simulink model "SRF_2DOF_Method"  (R2024b)
settings: Solver=VariableStepAuto  StartTime=0.0  StopTime=0.6  RelTol=1e-3
undefined symbols (not defined in the file): alpha, beta, ti
libraries: spsSeriesRLCBranchLib x6, spsMosfetLib x6, spsThreePhaseVIMeasurementLib x3, spsThreePhaseSeriesRLCBranchLib x2, eeGeneralControl x2, slpidlib x2, spsabctodq0Lib x2, spsCurrentMeasurementLib x1, spsGroundLib x1, spsdq0toabcLib x1, spsThreePhaseBreakerLib x1, spsThreePhaseSourceLib x1
settings Model: Creator=ASUS  LastModifiedBy=ASUS
settings DataIOCC: SaveFormat=StructureWithTime  ReturnWorkspaceOutputs=off

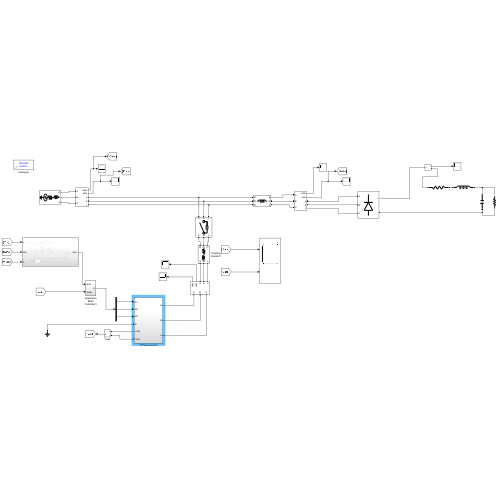
[thumbnail: Simulink's stored preview of the top-level diagram]
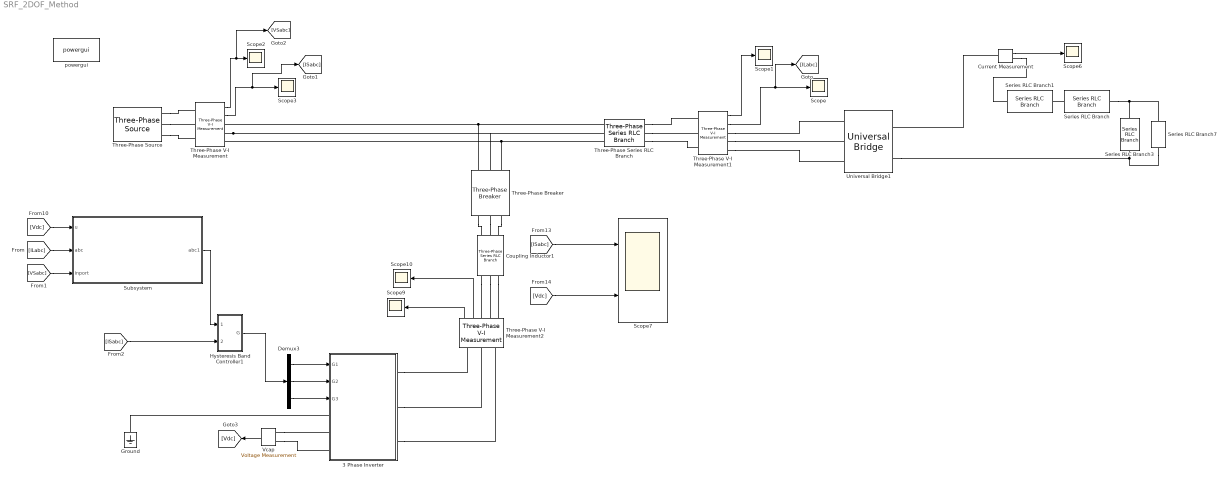
== system SRF_2DOF_Method ==
  3 Phase Inverter : Subsystem
  Coupling Inductor1 : spsThreePhaseSeriesRLCBranchLib/Three-Phase Series RLC Branch  LConnTagsString=A|B|C  RConnTagsString=A|B|C  BranchType=RL  Resistance=0.01  Inductance=3.5e-3  Capacitance=1e-6  Measurements=None
  Current Measurement : spsCurrentMeasurementLib/Current Measurement  PhasorSimulation=off  OutputType=Complex  PSBequivalent=0
  Demux3 : Demux  Outputs=3
  Ground : spsGroundLib/Ground  LConnTagsString=a
  Hysteresis Band Controller1 : Subsystem
  Scope{,1..3,6,9..10} (7 alike) : Scope
  Scope7 : Scope  NumInputPorts=2
  Series RLC Branch : spsSeriesRLCBranchLib/Series RLC Branch  LConnTagsString=__new0  RConnTagsString=__new0  BranchType=L  Resistance=50  Inductance=2e-6  SetiL0=off  InitialCurrent=0  Capacitance=1e-6  Setx0=off  InitialVoltage=0  Measurements=None
  Series RLC Branch1 : spsSeriesRLCBranchLib/Series RLC Branch  LConnTagsString=__new0  RConnTagsString=__new0  BranchType=R  Resistance=0.06  Inductance=1e-3  SetiL0=off  InitialCurrent=0  Capacitance=1e-6  Setx0=off  InitialVoltage=0  Measurements=None
  Series RLC Branch3 : spsSeriesRLCBranchLib/Series RLC Branch  LConnTagsString=__new0  RConnTagsString=__new0  BranchType=C  Resistance=50  Inductance=1e-3  SetiL0=off  InitialCurrent=0  Capacitance=3.63e-9  Setx0=off  InitialVoltage=0  Measurements=None
  Series RLC Branch7 : spsSeriesRLCBranchLib/Series RLC Branch  LConnTagsString=__new0  RConnTagsString=__new0  BranchType=R  Resistance=51.054  Inductance=1e-3  SetiL0=off  InitialCurrent=0  Capacitance=1e-6  Setx0=off  InitialVoltage=0  Measurements=None
  Subsystem : Subsystem
  Three-Phase Series RLC Branch : spsThreePhaseSeriesRLCBranchLib/Three-Phase Series RLC Branch  LConnTagsString=A|B|C  RConnTagsString=A|B|C  BranchType=L  Resistance=1  Inductance=1e-3  Capacitance=1e-6  Measurements=None
  Three-Phase V-I Measurement : spsThreePhaseVIMeasurementLib/Three-Phase V-I Measurement  VoltageMeasurement=phase-to-ground  SetLabelV=off  LabelV=Vabc  Vpu=off  VpuLL=off  CurrentMeasurement=yes  SetLabelI=off  LabelI=Iabc  Ipu=off  Pbase=100e6  Vbase=500e3  OutputType=Complex  PhasorSimulation=off  PSBequivalent=0
  Three-Phase V-I Measurement1 : spsThreePhaseVIMeasurementLib/Three-Phase V-I Measurement  VoltageMeasurement=phase-to-ground  SetLabelV=off  LabelV=Vabc  Vpu=off  VpuLL=off  CurrentMeasurement=yes  SetLabelI=off  LabelI=Iabc  Ipu=off  Pbase=100e6  Vbase=500e3  OutputType=Complex  PhasorSimulation=off  PSBequivalent=0
  Three-Phase V-I Measurement2 : spsThreePhaseVIMeasurementLib/Three-Phase V-I Measurement  VoltageMeasurement=phase-to-ground  SetLabelV=off  LabelV=Vabc  Vpu=off  VpuLL=off  CurrentMeasurement=yes  SetLabelI=off  LabelI=Iabc  Ipu=off  Pbase=100e6  Vbase=500e3  OutputType=Complex  PhasorSimulation=off  PSBequivalent=0
  Three-Phase Breaker : spsThreePhaseBreakerLib/Three-Phase Breaker  InitialState=open  SwitchA=on  SwitchB=on  SwitchC=on  SwitchTimes=[0.2 0.5]  External=off  BreakerResistance=0.01  SnubberResistance=1e6  SnubberCapacitance=inf  Measurements=None
  Three-Phase Source : spsThreePhaseSourceLib/Three-Phase Source  InternalConnection=Yg  VoltagePhases=off  Voltage=415  PhaseAngle=0  Voltage_phases=[25e3 25e3 25e3]/sqrt(3)  PhaseAngles_phases=[0 -120 +120]  Frequency=50  NonIdealSource=on  SpecifyImpedance=off  Resistance=0.86  Inductance=1e-4  ShortCircuitLevel=100e6  BaseVoltage=25e3  XRratio=7  BusType=swing  Pref=10e3  Qref=0  Prefabc=[10e3, 10e3, 10e3]  Qrefabc=[0, 0, 0]  Qmin=-inf  Qmax=inf
  Universal Bridge1 : spsUniversalBridgeLib/Universal Bridge  Arms=3  SnubberResistance=1e5  SnubberCapacitance=inf  Device=Diodes  Ron=1e-3  Lon=0  ForwardVoltages="[  0  0  ]"  ForwardVoltage=0  GTOparameters=[ 10e-6 , 20e-6 ]  IGBTparameters=[ 1e-6 , 2e-6 ]  Measurements=None  Measurements_2=None  converterType=Rectifier
  Vcap : spsVoltageMeasurementLib/Voltage Measurement  PhasorSimulation=off  OutputType=Complex  PSBequivalent=0
  powergui : spspowerguiLib/powergui  Priority=1  SimulationMode=Discrete  SampleTime=30e-07  frequency=60  Iterations=50  frequencyindice=0  Pbase=100e6  ErrMax=1e-4  UnitsV=kV  UnitsW=MW  buscounter=0  FunctionMessages=off  echomessages=off  EnableUseOfTLC=off  CurrentSourceSwitches=off  DisableSnubberDevices=off  DisableRonSwitches=off  DisableVfSwitches=off  DisplayEquations=off  AutomaticDiscreteSolvers=off  SolverType=Tustin/Backward Euler (TBE)  Interpol=off  ExternalGateDelay=off  methode=off  Ts=100  x0status=blocks  SPID=on  SwTol=0  HookPort=off  NonlinearTolerance=1e-4  nMaxIteration=100  ContinueOnMaxIteration=off  RestoreLinks=warning  ResistiveCurrentMeasurement=off  Frange=[0:2:500]  Ylog=off  Xlog=on  ShowGrid=off  save=off  variable=ZData  structure=0  ZoomFFT=off  StartTime=0.0  cycles=1  DisplayStyle=1  fundamental=60  FreqAxis=off  MaxFrequency=1000  frequencyindicesteady=1  RmsSteady=1  display=off
  wires:
  Demux3/3 -> 3 Phase Inverter/3(G3)
  Current Measurement/1 -> Scope6/1
  [Vdc] -> Scope7/2
  Three-Phase V-I Measurement/2 -> [ISabc], Scope3/1
  Three-Phase V-I Measurement1/2 -> [ILabc], Scope/1
  Demux3/2 -> 3 Phase Inverter/2(G2)
  Three-Phase V-I Measurement1/1 -> Scope1/1
  Three-Phase V-I Measurement/1 -> [VSabc], Scope2/1
  Hysteresis Band Controller1/1(G) -> Demux3/1
  [ISabc] -> Hysteresis Band Controller1/2(ISabc)
  Three-Phase V-I Measurement2/2 -> Scope10/1
  [ISabc] -> Scope7/1
  Demux3/1 -> 3 Phase Inverter/1(G1)
  Vcap/1 -> [Vdc]
  Three-Phase V-I Measurement2/1 -> Scope9/1
  [VSabc] -> Subsystem/3(Inport)
  [Vdc] -> Subsystem/1(u)
  [ILabc] -> Subsystem/2(abc)
  Subsystem/1(abc1) -> Hysteresis Band Controller1/1(Isref)
  connections:
  Universal Bridge1/RConn2 -- Series RLC Branch3/RConn1 -- Series RLC Branch7/RConn1
  Three-Phase Breaker/RConn1 -- Three-Phase V-I Measurement/RConn1 -- Three-Phase Series RLC Branch/LConn1
  Series RLC Branch/RConn1 -- Series RLC Branch3/LConn1 -- Series RLC Branch7/LConn1
  Three-Phase Breaker/RConn3 -- Three-Phase V-I Measurement/RConn3 -- Three-Phase Series RLC Branch/LConn3
  Three-Phase V-I Measurement/RConn2 -- Three-Phase Series RLC Branch/LConn2 -- Three-Phase Breaker/RConn2
  Three-Phase Series RLC Branch/RConn2 -- Three-Phase V-I Measurement1/LConn2
  Three-Phase Source/RConn2 -- Three-Phase V-I Measurement/LConn2
  Three-Phase Series RLC Branch/RConn1 -- Three-Phase V-I Measurement1/LConn1
  3 Phase Inverter/RConn3 -- Three-Phase V-I Measurement2/LConn3
  Coupling Inductor1/RConn2 -- Three-Phase V-I Measurement2/RConn2
  3 Phase Inverter/LConn1 -- Ground/LConn1
  Three-Phase Series RLC Branch/RConn3 -- Three-Phase V-I Measurement1/LConn3
  Vcap/LConn1 -- 3 Phase Inverter/LConn2
  Coupling Inductor1/RConn3 -- Three-Phase V-I Measurement2/RConn3
  3 Phase Inverter/RConn2 -- Three-Phase V-I Measurement2/LConn2
  Three-Phase Breaker/LConn2 -- Coupling Inductor1/LConn2
  Three-Phase Source/RConn1 -- Three-Phase V-I Measurement/LConn1
  Current Measurement/LConn1 -- Universal Bridge1/RConn1
  Three-Phase V-I Measurement1/RConn1 -- Universal Bridge1/LConn1
  Three-Phase V-I Measurement1/RConn2 -- Universal Bridge1/LConn2
  Three-Phase V-I Measurement1/RConn3 -- Universal Bridge1/LConn3
  Three-Phase Source/RConn3 -- Three-Phase V-I Measurement/LConn3
  Three-Phase Breaker/LConn3 -- Coupling Inductor1/LConn3
  Coupling Inductor1/RConn1 -- Three-Phase V-I Measurement2/RConn1
  Vcap/LConn2 -- 3 Phase Inverter/LConn3
  Current Measurement/RConn1 -- Series RLC Branch1/RConn1
  3 Phase Inverter/RConn1 -- Three-Phase V-I Measurement2/LConn1
  Three-Phase Breaker/LConn1 -- Coupling Inductor1/LConn1
  Series RLC Branch/LConn1 -- Series RLC Branch1/LConn1

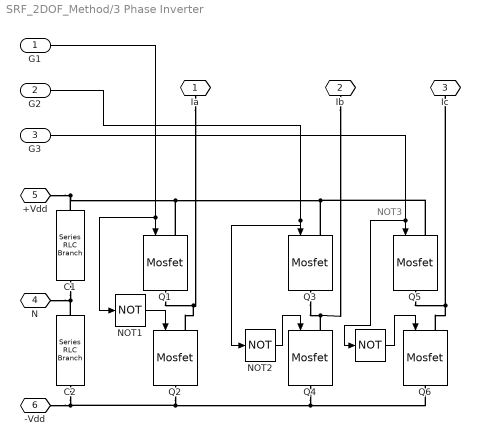
== system SRF_2DOF_Method/3 Phase Inverter ==
  note: NOT3
  G1 : Inport
  G2 : Inport  Port=2
  G3 : Inport  Port=3
  " " : Logic  Operator=NOT  AllPortsSameDT=off  OutDataTypeStr=boolean
  C1 : spsSeriesRLCBranchLib/Series RLC Branch  LConnTagsString=__new0  RConnTagsString=__new0  BranchType=C  Resistance=1  Inductance=1e-3  SetiL0=off  InitialCurrent=0  Capacitance=4700e-6  Setx0=off  InitialVoltage=350  Measurements=None
  C2 : spsSeriesRLCBranchLib/Series RLC Branch  LConnTagsString=__new0  RConnTagsString=__new0  BranchType=C  Resistance=1  Inductance=1e-3  SetiL0=off  InitialCurrent=0  Capacitance=4700e-6  Setx0=off  InitialVoltage=350  Measurements=None
  NOT1 : Logic  Operator=NOT  AllPortsSameDT=off  OutDataTypeStr=boolean
  NOT2 : Logic  Operator=NOT  AllPortsSameDT=off  OutDataTypeStr=boolean
  Q{1..6} (6 alike) : spsMosfetLib/Mosfet  Ron=0.01  Lon=0  Rd=0.01  Vfd=0  IC=0  Rs=1e10  Cs=inf  Measurements=off
  Ia : PMIOPort  Side=Right
  Ib : PMIOPort  Port=2  Side=Right
  Ic : PMIOPort  Port=3  Side=Right
  N : PMIOPort  Port=4  Side=Left
  +Vdd : PMIOPort  Port=5  Side=Left
  -Vdd : PMIOPort  Port=6  Side=Left
  wires:
  NOT1/1 -> Q2/1
  NOT2/1 -> Q4/1
  " "/1 -> Q6/1
  G1/1 -> NOT1/1, Q1/1
  G2/1 -> Q3/1, NOT2/1
  G3/1 -> Q5/1, " "/1
  connections:
  Q1/RConn1 -- Ia/RConn1 -- Q2/LConn1
  Q3/RConn1 -- Ib/RConn1 -- Q4/LConn1
  Q2/RConn1 -- C2/RConn1 -- -Vdd/RConn1 -- Q4/RConn1 -- Q6/RConn1
  Q6/LConn1 -- Ic/RConn1 -- Q5/RConn1
  C1/LConn1 -- Q1/LConn1 -- Q5/LConn1 -- Q3/LConn1 -- +Vdd/RConn1
  N/RConn1 -- C1/RConn1 -- C2/LConn1

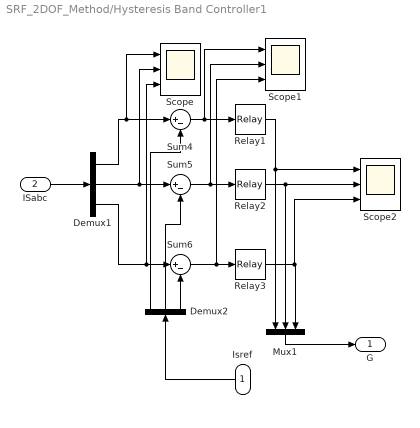
== system SRF_2DOF_Method/Hysteresis Band Controller1 ==
  Isref : Inport
  ISabc : Inport  Port=2
  Demux1 : Demux  Outputs=3
  Demux2 : Demux  Outputs=3
  Mux1 : Mux  Inputs=3
  Relay1 : Relay  OnSwitchValue=0.0001  OffSwitchValue=-0.0001  ZeroCross=off
  Relay2 : Relay  OnSwitchValue=0.0001  OffSwitchValue=-0.0001  ZeroCross=off
  Relay3 : Relay  OnSwitchValue=0.0001  OffSwitchValue=-0.0001  ZeroCross=off
  Scope : Scope  NumInputPorts=3
  Scope1 : Scope  NumInputPorts=3
  Scope2 : Scope  NumInputPorts=3
  Sum4 : Sum  Inputs=|+-
  Sum5 : Sum  Inputs=|+-
  Sum6 : Sum  Inputs=|+-
  G : Outport
  wires:
  Isref/1 -> Demux2/1
  ISabc/1 -> Demux1/1
  Mux1/1 -> G/1
  Sum4/1 -> Relay1/1, Scope1/1
  Demux2/1 -> Sum4/2
  Sum5/1 -> Relay2/1, Scope1/2
  Demux2/3 -> Sum6/2
  Demux1/3 -> Sum6/1, Scope/3
  Demux1/1 -> Sum4/1, Scope/1
  Sum6/1 -> Relay3/1, Scope1/3
  Demux1/2 -> Sum5/1, Scope/2
  Demux2/2 -> Sum5/2
  Relay2/1 -> Scope2/2, Mux1/2
  Relay1/1 -> Mux1/1, Scope2/1
  Relay3/1 -> Mux1/3, Scope2/3

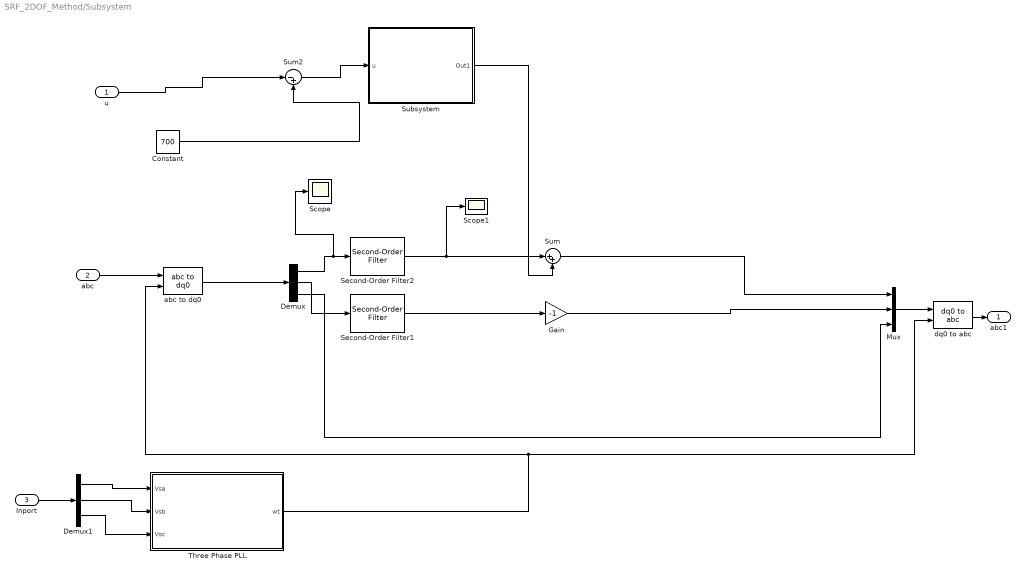
== system SRF_2DOF_Method/Subsystem ==
  u : Inport
  abc : Inport  Port=2
  Inport : Inport  Port=3
  Constant : Constant  Value=700
  Demux : Demux  Outputs=3
  Demux1 : Demux  Outputs=3
  Gain : Gain  Gain=-1
  Mux : Mux  Inputs=3
  Scope : Scope
  Scope1 : Scope
  Second-Order Filter1 : eeGeneralControl/Second-Order Filter  FilterType=Low-pass  fn=5  Zeta=0.707  Ts=-1  A0=0  Ph0=0  f0=0  b0=0
  Second-Order Filter2 : eeGeneralControl/Second-Order Filter  FilterType=Low-pass  fn=5  Zeta=0.707  Ts=-1  A0=0  Ph0=0  f0=0  b0=0
  Subsystem : Subsystem
  Sum : Sum  Inputs=|++
  Sum2 : Sum  Inputs=|-+
  Three Phase PLL : Subsystem
  abc to dq0 : spsabctodq0Lib/abc to dq0  Alignment=90 degrees behind phase A axis
  dq0 to abc : spsdq0toabcLib/dq0 to abc  Alignment=90 degrees behind phase A axis
  abc1 : Outport
  wires:
  Three Phase PLL/1(wt) -> dq0 to abc/2, abc to dq0/2
  Demux/2 -> Second-Order Filter1/1
  abc to dq0/1 -> Demux/1
  Subsystem/1(Out1) -> Sum/2
  Sum/1 -> Mux/1
  Second-Order Filter2/1 -> Scope1/1, Sum/1
  Second-Order Filter1/1 -> Gain/1
  Demux1/2 -> Three Phase PLL/2(Vsb)
  Demux/3 -> Mux/3
  Gain/1 -> Mux/2
  Mux/1 -> dq0 to abc/1
  Demux/1 -> Scope/1, Second-Order Filter2/1
  Demux1/3 -> Three Phase PLL/3(Vsc)
  dq0 to abc/1 -> abc1/1
  Constant/1 -> Sum2/2
  abc/1 -> abc to dq0/1
  Demux1/1 -> Three Phase PLL/1(Vsa)
  Inport/1 -> Demux1/1
  u/1 -> Sum2/1
  Sum2/1 -> Subsystem/1(u)

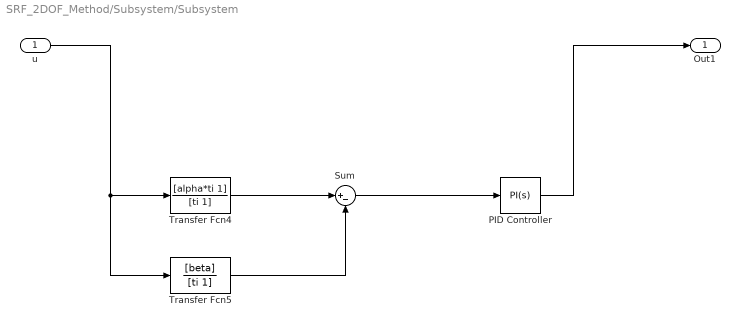
== system SRF_2DOF_Method/Subsystem/Subsystem ==
  u : Inport
  PID Controller : slpidlib/PID Controller  Controller=PI  Form=Parallel  TimeDomain=Continuous-time  UseExternalTs=off  SampleTime=-1  IntegratorMethod=Forward Euler  FilterMethod=Forward Euler  ControllerParametersSource=internal  P=0.5  I=0.009  UseKiTs=off  D=0  UseExternalDerivativeSource=off  N=100  UseFilter=on  TunerSelectOption=Transfer Function Based (PID Tuner App)  InitialConditionSource=internal  InitialConditionForIntegrator=0  InitialConditionForFilter=0  DifferentiatorICPrevScaledInput=0  ExternalReset=none  TrackingMode=off  Kt=1  LimitOutput=off  SatLimitsSource=internal  UpperSaturationLimit=inf  LowerSaturationLimit=-inf  LinearizeAsGain=on  AntiWindupMode=none  Kb=1  LimitIntegrator=off  UpperIntegratorSaturationLimit=inf  LowerIntegratorSaturationLimit=-inf  POutMin=[]  POutMax=[]  IOutMin=[]  IOutMax=[]  DOutMin=[]  DOutMax=[]  NOutMin=[]  NOutMax=[]  SumOutMin=[]  SumOutMax=[]  SaturationOutMin=[]  SaturationOutMax=[]  PParamMin=[]  PParamMax=[]  IParamMin=[]  IParamMax=[]  DParamMin=[]  DParamMax=[]  NParamMin=[]  NParamMax=[]  KbParamMin=[]  KbParamMax=[]  KtParamMin=[]  KtParamMax=[]  KbOutMin=[]  KbOutMax=[]  KtOutMin=[]  KtOutMax=[]  IntegratorOutMin=[]  IntegratorOutMax=[]  FilterOutMin=[]  FilterOutMax=[]  SumI1OutMin=[]  SumI1OutMax=[]  SumI2OutMin=[]  SumI2OutMax=[]  SumI3OutMin=[]  SumI3OutMax=[]  SumI4OutMin=[]  SumI4OutMax=[]  SumDOutMin=[]  SumDOutMax=[]  DifferentiatorOutMin=[]  DifferentiatorOutMax=[]  FilterDiffOutCoefMin=[]  FilterDiffOutCoefMax=[]  ReciprocalOutMin=[]  ReciprocalOutMax=[]  SumDenOutMin=[]  SumDenOutMax=[]  SumNumOutMin=[]  SumNumOutMax=[]  DivideOutMin=[]  DivideOutMax=[]  UdiffTsProdOutMin=[]  UdiffTsProdOutMax=[]  NTsProdOutMin=[]  NTsProdOutMax=[]  UintegralTsProdOutMin=[]  UintegralTsProdOutMax=[]  UngainTsProdOutMin=[]  UngainTsProdOutMax=[]  ClampingZeroOutDataTypeStr=Inherit: Inherit via back propagation  ClampingZeroOutMin=[]  ClampingZeroOutMax=[]  FilterDenConstantOutDataTypeStr=Inherit: Inherit via back propagation  FilterDenConstantOutMin=[]  FilterDenConstantOutMax=[]  PCopyOutDataTypeStr=Inherit: Inherit via back propagation  PCopyOutMin=[]  PCopyOutMax=[]  NCopyOutDataTypeStr=Inherit: Inherit via back propagation  NCopyOutMin=[]  NCopyOutMax=[]  IntegratorContinuousStateAttributes=''  IntegratorStateMustResolveToSignalObject=off  IntegratorRTWStateStorageClass=Auto  FilterContinuousStateAttributes=''  FilterStateMustResolveToSignalObject=off  FilterRTWStateStorageClass=Auto  ParallelPVariant=InternalParameters  IdealPVariant=Disabled  IVariant=InternalParameters  DVariant=Disabled  IntegratorVariant=Continuous  SatVariant=Disabled  AWVariant=Passthrough  PCopyVariant=Disabled  TRVariant=Disabled  FdbkBlocksVariant=Forward  IdealPFdbkVariant=Disabled  SatFdbkVariant=Disabled  DerivativeFilterVariant=Disabled  NVariant=Disabled  NCopyVariant=Disabled_SignalSpec  FilterICVariant=Disabled  IntegratorICVariant=InternalICs  ExternalResetVariant=Disabled  TRSumVariant=Passthrough  SumFdbkVariant=Disabled  SumVariant=Sum_PI  TsampFilterVariant=InternalTs  TsampNgainVariant=Passthrough  TsampIntegralVariant=Disabled_SignalSpec  ExternalSaturationOutDataTypeStr=Inherit: Same as second input  DerivativeSourceVariant=Disabled  PreIntVariant=InternalPreInt
  Sum : Sum  Inputs=|+-
  Transfer Fcn4 : TransferFcn  Numerator=[alpha*ti 1]  Denominator=[ti 1]
  Transfer Fcn5 : TransferFcn  Numerator=[beta]  Denominator=[ti 1]
  Out1 : Outport
  wires:
  Transfer Fcn4/1 -> Sum/1
  u/1 -> Transfer Fcn4/1, Transfer Fcn5/1
  Transfer Fcn5/1 -> Sum/2
  Sum/1 -> PID Controller/1
  PID Controller/1 -> Out1/1

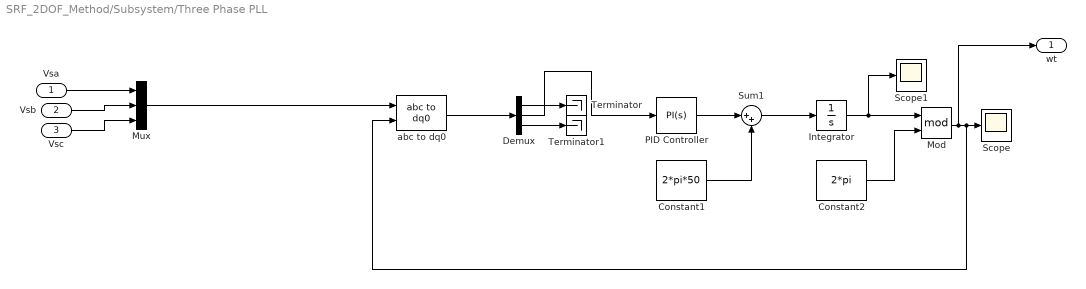
== system SRF_2DOF_Method/Subsystem/Three Phase PLL ==
  Vsa : Inport
  Vsb : Inport  Port=2
  Vsc : Inport  Port=3
  Constant1 : Constant  Value=2*pi*50
  Constant2 : Constant  Value=2*pi
  Demux : Demux  Outputs=3
  Integrator : Integrator
  Mod : Math  Operator=mod
  Mux : Mux  Inputs=3
  PID Controller : slpidlib/PID Controller  Controller=PI  Form=Parallel  TimeDomain=Continuous-time  UseExternalTs=off  SampleTime=3e-06  IntegratorMethod=Forward Euler  FilterMethod=Forward Euler  ControllerParametersSource=internal  P=430  I=0.6087  UseKiTs=off  D=0  UseExternalDerivativeSource=off  N=100  UseFilter=on  TunerSelectOption=Transfer Function Based (PID Tuner App)  InitialConditionSource=internal  InitialConditionForIntegrator=0  InitialConditionForFilter=0  DifferentiatorICPrevScaledInput=0  ExternalReset=none  TrackingMode=off  Kt=1  LimitOutput=off  SatLimitsSource=internal  UpperSaturationLimit=inf  LowerSaturationLimit=-inf  LinearizeAsGain=on  AntiWindupMode=none  Kb=1  LimitIntegrator=off  UpperIntegratorSaturationLimit=inf  LowerIntegratorSaturationLimit=-inf  POutMin=[]  POutMax=[]  IOutMin=[]  IOutMax=[]  DOutMin=[]  DOutMax=[]  NOutMin=[]  NOutMax=[]  SumOutMin=[]  SumOutMax=[]  SaturationOutMin=[]  SaturationOutMax=[]  PParamMin=[]  PParamMax=[]  IParamMin=[]  IParamMax=[]  DParamMin=[]  DParamMax=[]  NParamMin=[]  NParamMax=[]  KbParamMin=[]  KbParamMax=[]  KtParamMin=[]  KtParamMax=[]  KbOutMin=[]  KbOutMax=[]  KtOutMin=[]  KtOutMax=[]  IntegratorOutMin=[]  IntegratorOutMax=[]  FilterOutMin=[]  FilterOutMax=[]  SumI1OutMin=[]  SumI1OutMax=[]  SumI2OutMin=[]  SumI2OutMax=[]  SumI3OutMin=[]  SumI3OutMax=[]  SumI4OutMin=[]  SumI4OutMax=[]  SumDOutMin=[]  SumDOutMax=[]  DifferentiatorOutMin=[]  DifferentiatorOutMax=[]  FilterDiffOutCoefMin=[]  FilterDiffOutCoefMax=[]  ReciprocalOutMin=[]  ReciprocalOutMax=[]  SumDenOutMin=[]  SumDenOutMax=[]  SumNumOutMin=[]  SumNumOutMax=[]  DivideOutMin=[]  DivideOutMax=[]  UdiffTsProdOutMin=[]  UdiffTsProdOutMax=[]  NTsProdOutMin=[]  NTsProdOutMax=[]  UintegralTsProdOutMin=[]  UintegralTsProdOutMax=[]  UngainTsProdOutMin=[]  UngainTsProdOutMax=[]  ClampingZeroOutDataTypeStr=Inherit: Inherit via back propagation  ClampingZeroOutMin=[]  ClampingZeroOutMax=[]  FilterDenConstantOutDataTypeStr=Inherit: Inherit via back propagation  FilterDenConstantOutMin=[]  FilterDenConstantOutMax=[]  PCopyOutDataTypeStr=Inherit: Inherit via back propagation  PCopyOutMin=[]  PCopyOutMax=[]  NCopyOutDataTypeStr=Inherit: Inherit via back propagation  NCopyOutMin=[]  NCopyOutMax=[]  IntegratorContinuousStateAttributes=''  IntegratorStateMustResolveToSignalObject=off  IntegratorRTWStateStorageClass=Auto  FilterContinuousStateAttributes=''  FilterStateMustResolveToSignalObject=off  FilterRTWStateStorageClass=Auto  ParallelPVariant=InternalParameters  IdealPVariant=Disabled  IVariant=InternalParameters  DVariant=Disabled  IntegratorVariant=Continuous  SatVariant=Disabled  AWVariant=Passthrough  PCopyVariant=Disabled  TRVariant=Disabled  FdbkBlocksVariant=Forward  IdealPFdbkVariant=Disabled  SatFdbkVariant=Disabled  DerivativeFilterVariant=Disabled  NVariant=Disabled  NCopyVariant=Disabled_SignalSpec  FilterICVariant=Disabled  IntegratorICVariant=InternalICs  ExternalResetVariant=Disabled  TRSumVariant=Passthrough  SumFdbkVariant=Disabled  SumVariant=Sum_PI  TsampFilterVariant=InternalTs  TsampNgainVariant=Passthrough  TsampIntegralVariant=Disabled_SignalSpec  ExternalSaturationOutDataTypeStr=Inherit: Same as second input  DerivativeSourceVariant=Disabled  PreIntVariant=InternalPreInt
  Scope : Scope
  Scope1 : Scope
  Sum1 : Sum  Inputs=|++
  Terminator : Terminator
  Terminator1 : Terminator
  abc to dq0 : spsabctodq0Lib/abc to dq0  Alignment=90 degrees behind phase A axis
  wt : Outport
  wires:
  Constant2/1 -> Mod/2
  PID Controller/1 -> Sum1/1
  Mod/1 -> wt/1, abc to dq0/2, Scope/1
  Mux/1 -> abc to dq0/1
  Sum1/1 -> Integrator/1
  Integrator/1 -> Scope1/1, Mod/1
  Constant1/1 -> Sum1/2
  Demux/2 -> PID Controller/1
  Demux/1 -> Terminator/1
  Demux/3 -> Terminator1/1
  abc to dq0/1 -> Demux/1
  Vsa/1 -> Mux/1
  Vsb/1 -> Mux/2
  Vsc/1 -> Mux/3
